simulink model "rocket_tvc"  (R2025b)
settings: Solver=ode4  StartTime=0.0  StopTime=13  FixedStep=0.001  RelTol=1e-3
values from neighbouring files (symbols this model uses):
  BV = nz.b    [launch_model.m]
  NZ = nz.n    [launch_model.m]
  P = rocket_params()    [compare_simulink_vs_script.m]    (also in export_for_python.m; launch_model.m; run_nominal.m; study_montecarlo.m = base)
  X0 = [0; 0; 0;  0; 0; 0;  q0;  0; 0; 0;  0; 0]    [initial_state.m]    (also in launch_model.m = initial_state(P))
settings Model: Creator=Admin  LastModifiedBy=Admin
settings DataIOCC: SaveOutput=off  SignalLogging=off  SaveTime=off

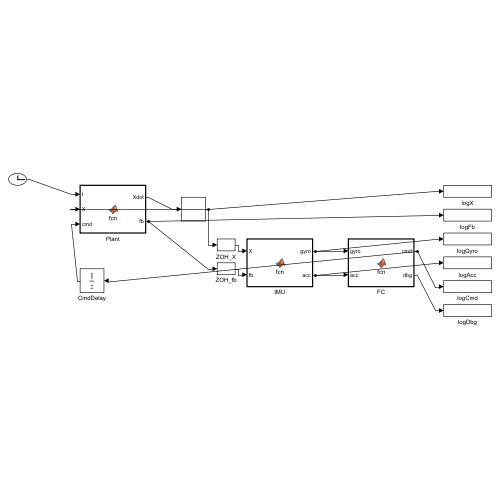
[thumbnail: Simulink's stored preview of the top-level diagram]
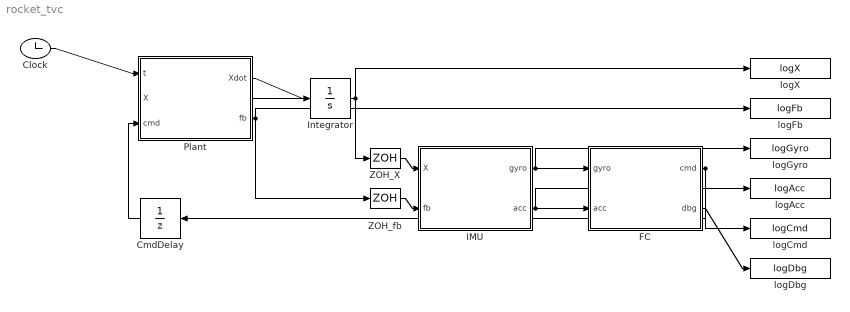
== system rocket_tvc ==
  Clock : Clock
  CmdDelay : UnitDelay  InitialCondition=zeros(2,1)  SampleTime=0.01  HasFrameUpgradeWarning=on
  FC : MATLAB Function  TreatAsAtomicUnit=on
  IMU : MATLAB Function  TreatAsAtomicUnit=on
  Integrator : Integrator  InitialCondition=X0
  Plant : MATLAB Function  TreatAsAtomicUnit=on
  ZOH_X : ZeroOrderHold  SampleTime=0.01
  ZOH_fb : ZeroOrderHold  SampleTime=0.01
  logAcc : ToWorkspace  VariableName=logAcc  SaveFormat=Timeseries  SampleTime=-1
  logCmd : ToWorkspace  VariableName=logCmd  SaveFormat=Timeseries  SampleTime=-1
  logDbg : ToWorkspace  VariableName=logDbg  SaveFormat=Timeseries  SampleTime=-1
  logFb : ToWorkspace  VariableName=logFb  SaveFormat=Timeseries  SampleTime=-1
      settings: Decimation=10
  logGyro : ToWorkspace  VariableName=logGyro  SaveFormat=Timeseries  SampleTime=-1
  logX : ToWorkspace  VariableName=logX  SaveFormat=Timeseries  SampleTime=-1
      settings: Decimation=10
  wires:
  Clock/1 -> Plant/1(t)
  Integrator/1 -> Plant/2(X), ZOH_X/1, logX/1
  CmdDelay/1 -> Plant/3(cmd)
  Plant/1(Xdot) -> Integrator/1
  Plant/2(fb) -> ZOH_fb/1, logFb/1
  ZOH_X/1 -> IMU/1(X)
  ZOH_fb/1 -> IMU/2(fb)
  IMU/1(gyro) -> FC/1(gyro), logGyro/1
  IMU/2(acc) -> FC/2(acc), logAcc/1
  FC/1(cmd) -> CmdDelay/1, logCmd/1
  FC/2(dbg) -> logDbg/1

== matlab function rocket_tvc/IMU ==
  data: X input; gyro output; fb input; acc output; P parameter; NZ parameter; BV parameter
function [gyro, acc] = fcn(X, fb, P, NZ, BV)
persistent k
if isempty(k), k = 0; end
[gyro, acc] = imu_model(X(11:13), fb, NZ(k+1, :), BV, P);
k = k + 1;

== matlab function rocket_tvc/Plant ==
  data: t input; Xdot output; X input; cmd input; fb output; P parameter
function [Xdot, fb] = fcn(t, X, cmd, P)
[Xdot, fb] = plant_deriv(t, X, cmd, P);

== matlab function rocket_tvc/FC ==
  data: gyro input; cmd output; acc input; dbg output; P parameter
function [cmd, dbg] = fcn(gyro, acc, P)
[cmd, dbg] = flight_computer(gyro, acc, P);
